simulink model "DahlinModel_Student"  (R2024b)
settings: Solver=VariableStepAuto  StartTime=0.0  StopTime=0.5  RelTol=1e-3
values from neighbouring files (symbols this model uses):
  b = 0.000498967    [Lez_11_DahlinModel_Parameters_Student.m]
  Bz_coeff = Bz{1,1}    [Lez_11_DahlinModel_Parameters_Student.m]
  Dz = minreal(Dz)    [Lez_11_DahlinModel_Parameters_Student.m]
  FFeedNum = Fz.Numerator{1,1}    [Lez_11_DahlinModel_Parameters_Student.m]
  Fz = Kf*(z-0.95)*(z-0.8)*z    [Lez_11_DahlinModel_Parameters_Student.m]
  J = 8.1035e-5    (= 8.1035e-05)    [Lez_11_DahlinModel_Parameters_Student.m]
  Km = 0.11    [Lez_11_DahlinModel_Parameters_Student.m]
  L = 0.0061    [Lez_11_DahlinModel_Parameters_Student.m]
  PulseNumber = 2048*4    (= 8192)    [Lez_11_DahlinModel_Parameters_Student.m]
  R = 3.1532    [Lez_11_DahlinModel_Parameters_Student.m]
  RadiantsPerCount = 2*pi/(PulseNumber-1)    (= 0.00076708403213)    [Lez_11_DahlinModel_Parameters_Student.m]
  RpmToRads = 2*pi/60    (= 0.10471975512)    [Lez_11_DahlinModel_Parameters_Student.m]
  TaoFilterOmega = 0.002    [Lez_11_DahlinModel_Parameters_Student.m]
  TSample = 0.1e-3    (= 0.0001)    [Lez_11_DahlinModel_Parameters_Student.m]
undefined symbols (not defined in the file or in its folder): DiscIntNeverNeededParam, dspblkCoreblockFVToolHelper, gcbh
settings Model: Creator=Davide  LastModifiedBy=andrea.gallo13
settings DataIOCC: ReturnWorkspaceOutputs=off
settings RTWCC: GPUComputeCapability=3.5

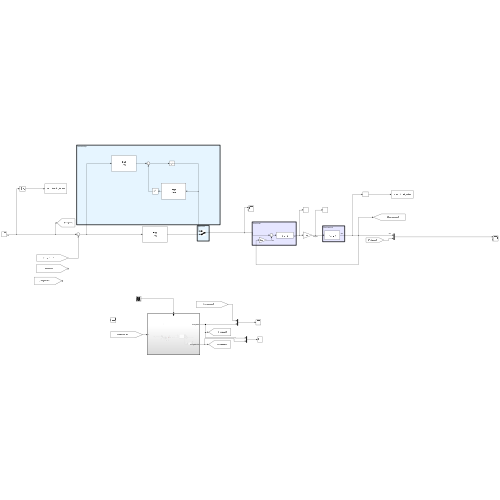
[thumbnail: Simulink's stored preview of the top-level diagram]
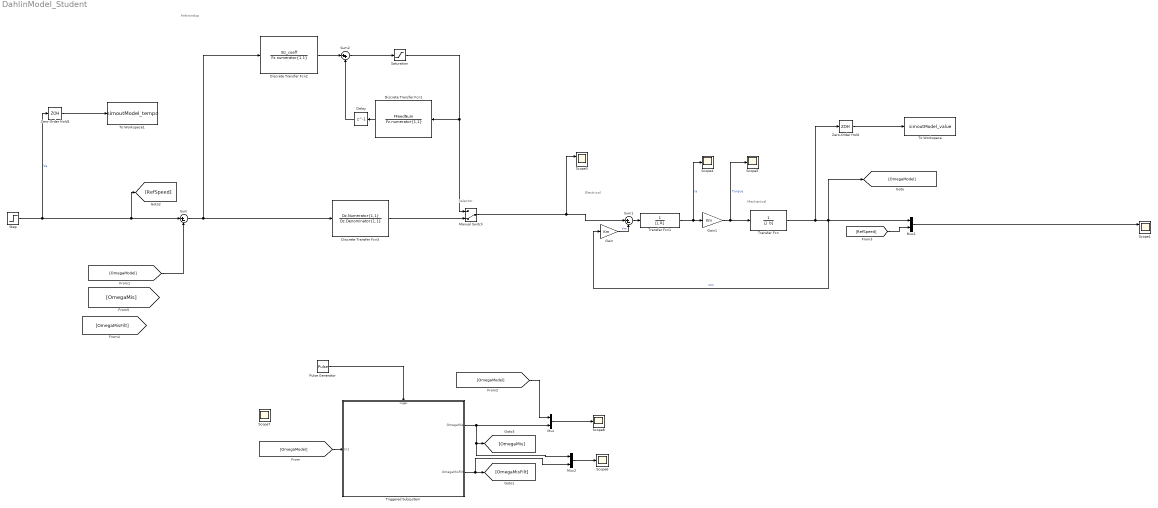
== system DahlinModel_Student ==
  note: Selector
  note: Antiwindup
  note: Mechanical
  note: Electrical
  Delay : Delay  DelayLength=1  InputProcessing=Columns as channels (frame based)
  Discrete Transfer Fcn1 : DiscreteTransferFcn  LoadFcn=dspblkCoreblockFVToolHelper(gcbh,'load');  Numerator=FFeedNum  Denominator=Fz.numerator{1,1}  SampleTime=TSample
      settings: CopyFcn=dspblkCoreblockFVToolHelper(gcbh,'copy');  DeleteFcn=dspblkCoreblockFVToolHelper(gcbh,'close');  ModelCloseFcn=dspblkCoreblockFVToolHelper(gcbh,'close');  PreSaveFcn=dspblkCoreblockFVToolHelper(gcbh,'presave');  PostSaveFcn=dspblkCoreblockFVToolHelper(gcbh,'postsave');  CloseFcn=dspblkCoreblockFVToolHelper(gcbh,'close');
  Discrete Transfer Fcn2 : DiscreteTransferFcn  LoadFcn=dspblkCoreblockFVToolHelper(gcbh,'load');  Numerator=Bz_coeff  Denominator=Fz.numerator{1,1}  SampleTime=TSample
      settings: CopyFcn=dspblkCoreblockFVToolHelper(gcbh,'copy');  DeleteFcn=dspblkCoreblockFVToolHelper(gcbh,'close');  ModelCloseFcn=dspblkCoreblockFVToolHelper(gcbh,'close');  PreSaveFcn=dspblkCoreblockFVToolHelper(gcbh,'presave');  PostSaveFcn=dspblkCoreblockFVToolHelper(gcbh,'postsave');  CloseFcn=dspblkCoreblockFVToolHelper(gcbh,'close');
  Discrete Transfer Fcn3 : DiscreteTransferFcn  LoadFcn=dspblkCoreblockFVToolHelper(gcbh,'load');  Numerator=Dz.Numerator{1,1}  Denominator=Dz.Denominator{1,1}  SampleTime=TSample
      settings: CopyFcn=dspblkCoreblockFVToolHelper(gcbh,'copy');  DeleteFcn=dspblkCoreblockFVToolHelper(gcbh,'close');  ModelCloseFcn=dspblkCoreblockFVToolHelper(gcbh,'close');  PreSaveFcn=dspblkCoreblockFVToolHelper(gcbh,'presave');  PostSaveFcn=dspblkCoreblockFVToolHelper(gcbh,'postsave');  CloseFcn=dspblkCoreblockFVToolHelper(gcbh,'close');
  Gain : Gain  Gain=Km
  Gain1 : Gain  Gain=Km
  Manual Switch : ManualSwitch  CurrentSetting=0
  Mux : Mux  Inputs=2
  Mux1 : Mux  Inputs=2
  Mux2 : Mux  Inputs=2
  Pulse Generator : DiscretePulseGenerator  PulseType=Time based  Period=TSample  PulseWidth=50
  Saturation : Saturate  UpperLimit=32  LowerLimit=-32
  Scope1 : Scope  NumInputPorts=3
  Scope3 : Scope  NumInputPorts=2
  Scope{4..8} (5 alike) : Scope
  Step : Step  Time=0  After=100  SampleTime=TSample
  Sum : Sum  Inputs=|+-
  Sum1 : Sum  Inputs=|+-
  Sum2 : Sum  Inputs=|++
  To Workspace : ToWorkspace  VariableName=simoutModel_value  SampleTime=-1
  To Workspace1 : ToWorkspace  VariableName=simoutModel_tempo  SampleTime=-1
  Transfer Fcn : TransferFcn  Denominator="[J  b]"
  Transfer Fcn1 : TransferFcn  Denominator=[L R]
  Triggered Subsystem : Subsystem  TreatAsAtomicUnit=on
  Zero-Order Hold : ZeroOrderHold  SampleTime=TSample
  Zero-Order Hold1 : ZeroOrderHold  SampleTime=TSample
  wires:
  Transfer Fcn/1 -> Zero-Order Hold/1, Gain/1, Mux1/1, [OmegaModel]  "wm"
  Gain/1 -> Sum1/2  "Vm"
  Gain1/1 -> Scope5/1, Transfer Fcn/1  "Torque"
  Sum1/1 -> Transfer Fcn1/1
  Transfer Fcn1/1 -> Scope4/1, Gain1/1  "ia"
  Step/1 -> Zero-Order Hold1/1, Sum/1, [RefSpeed]  "Va"
  Sum/1 -> Discrete Transfer Fcn2/1, Discrete Transfer Fcn3/1
  Pulse Generator/1 -> Triggered Subsystem/Trigger
  Mux/1 -> Scope8/1
  Manual Switch/1 -> Scope3/1, Sum1/1
  Triggered Subsystem/1(OmegaMis) -> Mux2/1, [OmegaMis], Mux/2
  [OmegaModel] -> Triggered Subsystem/1(In1)
  [OmegaModel] -> Mux/1
  Triggered Subsystem/2(OmegaMisFilt) -> Mux2/2, [OmegaMisFilt]
  Mux1/1 -> Scope1/1
  [RefSpeed] -> Mux1/2
  Discrete Transfer Fcn3/1 -> Manual Switch/2
  Mux2/1 -> Scope6/1
  Zero-Order Hold/1 -> To Workspace/1
  [OmegaModel] -> Sum/2
  Discrete Transfer Fcn2/1 -> Sum2/1
  Sum2/1 -> Saturation/1
  Saturation/1 -> Discrete Transfer Fcn1/1, Manual Switch/1
  Discrete Transfer Fcn1/1 -> Delay/1
  Delay/1 -> Sum2/2
  Zero-Order Hold1/1 -> To Workspace1/1

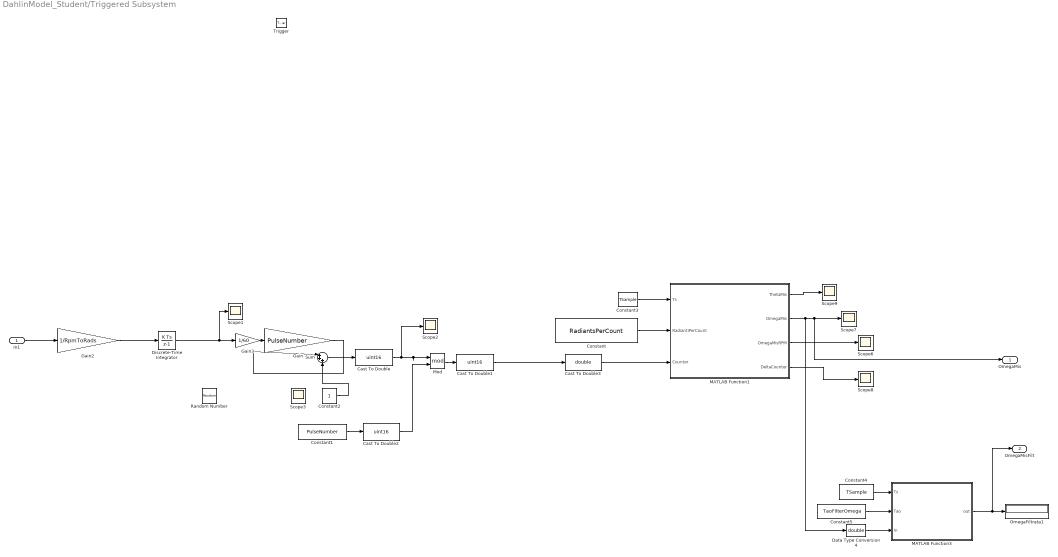
== system DahlinModel_Student/Triggered Subsystem ==
  In1 : Inport
  Trigger : TriggerPort  VariantControl=(inherit)
  Cast To Double : DataTypeConversion  OutDataTypeStr=uint16  SaturateOnIntegerOverflow=off  RndMeth=Floor
  Cast To Double1 : DataTypeConversion  OutDataTypeStr=uint16  SaturateOnIntegerOverflow=off  RndMeth=Floor
  Cast To Double2 : DataTypeConversion  OutDataTypeStr=uint16  SaturateOnIntegerOverflow=off  RndMeth=Floor
  Cast To Double3 : DataTypeConversion  OutDataTypeStr=double  SaturateOnIntegerOverflow=off  RndMeth=Floor
  Constant : Constant  Value=RadiantsPerCount
  Constant1 : Constant  Value=PulseNumber
  Constant2 : Constant
  Constant3 : Constant  Value=TSample
  Constant4 : Constant  Value=TSample  OutDataTypeStr=double
  Constant5 : Constant  Value=TaoFilterOmega  OutDataTypeStr=double
  Data Type Conversion4 : DataTypeConversion  OutDataTypeStr=double  SaturateOnIntegerOverflow=off  RndMeth=Floor
  Discrete-Time Integrator : DiscreteIntegrator  SampleTime=-1  ICPrevOutput=DiscIntNeverNeededParam  ICPrevScaledInput=DiscIntNeverNeededParam
  Gain : Gain  Gain=PulseNumber
  Gain2 : Gain  Gain=1/RpmToRads
  Gain3 : Gain  Gain=1/60
  MATLAB Function1 : MATLAB Function  TreatAsAtomicUnit=on
  MATLAB Function3 : MATLAB Function  TreatAsAtomicUnit=on
  Mod : Math  Operator=mod
  OmegaFiltrata1 : Display
  Random Number : RandomNumber  Variance=0.3
  Scope{1..3,6..9} (7 alike) : Scope
  Sum : Sum  Inputs=|+++
  OmegaMis : Outport
  OmegaMisFilt : Outport  Port=2
  wires:
  Cast To Double2/1 -> Mod/2
  Cast To Double/1 -> Scope2/1, Mod/1
  Constant1/1 -> Cast To Double2/1
  Mod/1 -> Cast To Double1/1
  Cast To Double1/1 -> Cast To Double3/1
  Gain/1 -> Sum/1
  Constant/1 -> MATLAB Function1/2(RadiantiPerCount)
  Constant3/1 -> MATLAB Function1/1(Ts)
  MATLAB Function1/3(OmegaMisRPM) -> Scope6/1
  Cast To Double3/1 -> MATLAB Function1/3(Counter)
  MATLAB Function1/1(ThetaMis) -> Scope9/1
  MATLAB Function1/2(OmegaMis) -> Data Type Conversion4/1, OmegaMis/1, Scope7/1
  MATLAB Function1/4(DeltaCounter) -> Scope8/1
  Gain3/1 -> Gain/1
  In1/1 -> Gain2/1
  Sum/1 -> Cast To Double/1
  Constant2/1 -> Sum/3
  Data Type Conversion4/1 -> MATLAB Function3/3(In)
  MATLAB Function3/1(out) -> OmegaMisFilt/1, OmegaFiltrata1/1
  Constant5/1 -> MATLAB Function3/2(Tao)
  Constant4/1 -> MATLAB Function3/1(Ts)
  Gain2/1 -> Discrete-Time Integrator/1
  Discrete-Time Integrator/1 -> Scope1/1, Gain3/1

== matlab function DahlinModel_Student/Triggered Subsystem/MATLAB Function3 ==
  data: Ts input; out output; Tao input; In input
function out  = LowPassFilter(  Ts ,Tao, In)

persistent OutPrecedente
if isempty( OutPrecedente )
    OutPrecedente = 0 ;
end    


    %Filtro passa basso discretizzato con il metodo delle differenze
    %all'indietro
    
    a=Ts/(Ts+Tao);
    b=Tao/(Ts+Tao);
    
    out=a*In+OutPrecedente*b;
   
    OutPrecedente = out;
   
end

== matlab function DahlinModel_Student/Triggered Subsystem/MATLAB Function1 ==
  data: Ts input; ThetaMis output; RadiantiPerCount input; Counter input; OmegaMis output; OmegaMisRPM output; DeltaCounter output
function [ThetaMis, OmegaMis, OmegaMisRPM, DeltaCounter] = CounterToThetaOmega(Ts, RadiantiPerCount, Counter)

% Inizializzazione dei valori iniziali 
persistent CounterPrec  
if isempty( CounterPrec )
    CounterPrec = 0;
end 

    DeltaCounter=Counter-CounterPrec;
    
    if (DeltaCounter>double(0x1000))
        DeltaCounter=DeltaCounter-double(0x2000);
    end
    
    if (DeltaCounter<-double(0x1000))
        DeltaCounter=DeltaCounter+double(0x2000);
    end
        
    % conversione conteggio in radianti
    ThetaMis = Counter * RadiantiPerCount;
    
    DeltaThetaMis = DeltaCounter*RadiantiPerCount;
   
    OmegaMis = DeltaThetaMis/Ts;
    OmegaMisRPM=OmegaMis*60/(2*pi);
 
    CounterPrec= Counter;
end
